simulink library "WECSim_Lib_Body_Elements"  (R2020b)
settings: Solver=VariableStepAuto  StartTime=0.0  StopTime=10.0  RelTol=1e-3
undefined symbols (not defined in the file or in its folder): body, simu, waves, X, Y, Z
libraries: nesl_utility x22, sm_lib x16, $bdroot x9, vrlib x3
(part 4 of 5)

== system WECSim_Lib_Body_Elements/Rigid Body/Hydrodynamic Body/Hydrostatic Restoring Force Calculation/Linear and Nonlinear Restoring Force Variant Subsystem/Linear Hydrostatic Restoring Force ==
  note: The total hydrostatic restoring force is due to a linear stiffness, the vertical buoyancy force (gravity - buoyancy) and a rotational buoyancy force if the center of gravity is not aligned with the center of buoyancy.
      |
      | F_restoring = F_linearRestoringStiffness + F_NetBuoyancy
      |
      | F_linear restoring = hydrostatic restoring coefficient * displacement
      | F_NetBuoyancy = F_gravity - F_buoyancy + F_rotational_buoyancy
      |
      | F_rotational_buoyancy = (cb-cg) x F_buoyancy
      | F_buoyancy = rho*g*V_0
      | F_gravity = m*g
  In1 : Inport
  Add : Sum
  Bus Selector : BusSelector  OutputSignals=mass,volume,centerBuoyancy,linearHydroRestCoef
  Net Buoyancy Force : Subsystem
  Product2 : Product  Multiplication=Matrix(*)
  Out1 : Outport
  wires:
  In1/1 -> Product2/2  "x"
  Bus Selector/4 -> Product2/1  "<linearHydroRestCoef>"
  Add/1 -> Out1/1  "F_Restoring"
  Product2/1 -> Add/2  "Linear Restoring Force"
  Net Buoyancy Force/1(F_NetBuoyancy) -> Add/1  "Net buoyancy force"
  [body1_hydroForce] -> Bus Selector/1
  Bus Selector/3 -> Net Buoyancy Force/3(Center of Buoyancy)  "<centerBuoyancy>"
  Bus Selector/2 -> Net Buoyancy Force/2(Volume)  "<volume>"
  Bus Selector/1 -> Net Buoyancy Force/1(Body Mass)  "<mass>"

== system WECSim_Lib_Body_Elements/Rigid Body/Hydrodynamic Body/Hydrostatic Restoring Force Calculation/Linear and Nonlinear Restoring Force Variant Subsystem/Nonlinear Hydrostatic Restoring Force ==
  In1 : Inport
  In2 : Inport  Port=2
  Bus Selector : BusSelector  OutputSignals=mass
  Center of Gravity : Constant  Value=body.centerGravity
  Gravity2 : Constant  Value=simu.gravity
  Rate Transition : RateTransition
  Rate Transition1 : RateTransition
  Restoring Forces : MATLAB Function  TreatAsAtomicUnit=on  SystemSampleTime=simu.nonlinearDt
  STL areas : Constant  Value=body.geometry.area
  STL centers : Constant  Value=body.geometry.center
  STL normal vectors : Constant  Value=body.geometry.norm
  To Workspace1 : ToWorkspace  VariableName=body1_hspressure_out  SaveFormat=Structure With Time  SampleTime=-1
      settings: Decimation=round(simu.dtOut/simu.dt,0)
  Water Density1 : Constant  Value=simu.rho
  Out1 : Outport
  wires:
  In1/1 -> Restoring Forces/1(x)
  Center of Gravity/1 -> Restoring Forces/8(cg)
  Gravity2/1 -> Restoring Forces/7(g)  "g"
  Water Density1/1 -> Restoring Forces/6(rho)
  STL normal vectors/1 -> Restoring Forces/4(tnorm)
  STL centers/1 -> Restoring Forces/3(center)
  In2/1 -> Restoring Forces/2(elv)
  STL areas/1 -> Restoring Forces/5(area)
  Bus Selector/1 -> Restoring Forces/9(mass)  "<mass>"
  Restoring Forces/2(p) -> Rate Transition1/1
  Rate Transition1/1 -> To Workspace1/1
  Restoring Forces/1(f) -> Rate Transition/1
  Rate Transition/1 -> Out1/1
  [body1_hydroForce] -> Bus Selector/1

== system WECSim_Lib_Body_Elements/Rigid Body/Hydrodynamic Body/Morison Element and Viscous Damping Force Calculation/Morison Element Variant Subsystem/Morison Element Off ==
  Constant : Constant  Value=zeros(1,body.dof)
  morison_force : Outport
  wires:
  Constant/1 -> morison_force/1

== system WECSim_Lib_Body_Elements/Rigid Body/Hydrodynamic Body/Morison Element and Viscous Damping Force Calculation/Morison Element Variant Subsystem/Morison Element On ==
  note: Chooses the appropriate Morison element variant dependent on the wave type. Note that if passive yaw is used, no block is chosen.
      |
      | If wave.type == 'noWave' | 'noWaveCIC' use No Wave Morison element
      | If wave.type == 'regularWave' | 'regularWaveCIC' use Regular Wave Morison element
      | If wave.type == 'irregularWave' or 'spectrumImport' use Irregular Wave Morison element
  note: 1) Add Subsystem or Model blocks as valid variant choices.
      | 2) You cannot connect blocks at this level. At simulation, connectivity is automatically
      | determined, based on the active variant and port name matching.
  displacement : Inport
  velocity : Inport  Port=2
  acceleration : Inport  Port=3
  time : Inport  Port=4
  Irregular Wave Morison Force : Subsystem  TreatAsAtomicUnit=on  SystemSampleTime=simu.morisonDt  VariantControl=sv_irregularWaves_b1
  No Wave Morison Force : Subsystem  VariantControl=sv_noWave
  Regular Wave Morison Force : Subsystem  TreatAsAtomicUnit=on  SystemSampleTime=simu.morisonDt  VariantControl=sv_regularWaves_b1
  morison_force : Outport

== system WECSim_Lib_Body_Elements/Rigid Body/Hydrodynamic Body/Nonlinear Wave Elevation/Linear or Instantaneous Free Surface/Instantaneous Water Free Surface ==
  note: Calculate the instantaneous wave elevation for the nonlinear hydrodynamics options.
  In1 : Inport
  In2 : Inport  Port=2
  Center of Gravity : Constant  Value=body.centerGravity
  Frequency Spacing : Constant  Value=waves.dOmega
  Instantaneous FS : MATLAB Function  TreatAsAtomicUnit=on
  Ramp Time : Constant  Value=simu.rampTime
  STL Centers : Constant  Value=body.geometry.center
  Wave Amplitude : Constant  Value=waves.amplitude
  Wave Direction : Constant  Value=waves.direction
  Wave Frequency : Constant  Value=waves.omega
  Wave Number : Constant  Value=waves.wavenumber
  Wave Random Phase : Constant  Value=waves.phase
  Wave Spread : Constant  Value=waves.spread
  Wave Type Number : Constant  Value=waves.typeNum
  Out1 : Outport
  wires:
  Instantaneous FS/1(f) -> Out1/1
  STL Centers/1 -> Instantaneous FS/2(center)
  Center of Gravity/1 -> Instantaneous FS/3(cg)
  Wave Number/1 -> Instantaneous FS/7(k)
  Wave Frequency/1 -> Instantaneous FS/5(w)
  Wave Type Number/1 -> Instantaneous FS/8(typeNum)
  Ramp Time/1 -> Instantaneous FS/10(rampT)
  Wave Random Phase/1 -> Instantaneous FS/11(phaseRand)
  Frequency Spacing/1 -> Instantaneous FS/6(dw)
  In2/1 -> Instantaneous FS/9(t)
  In1/1 -> Instantaneous FS/1(x)
  Wave Direction/1 -> Instantaneous FS/12(waveDir)
  Wave Amplitude/1 -> Instantaneous FS/4(AH)
  Wave Spread/1 -> Instantaneous FS/13(spread)

== system WECSim_Lib_Body_Elements/Rigid Body/Hydrodynamic Body/Nonlinear Wave Elevation/Linear or Instantaneous Free Surface/Mean Water Free Surface ==
  note: The mean water surface is always zero.
  zero : Constant  Value=0
  Out1 : Outport
  wires:
  zero/1 -> Out1/1

== system WECSim_Lib_Body_Elements/Rigid Body/Hydrodynamic Body/Variable Hydrodynamics Control/Variable Hydrodynamics Subsystem/noVariableHydro ==
  all_hydroForce : Inport
  Bus Selector : BusSelector  OutputSignals=hf1
  selected_hydroForce : Outport
  wires:
  Bus Selector/1 -> selected_hydroForce/1  "<hf1>"
  all_hydroForce/1 -> Bus Selector/1  "x"

== system WECSim_Lib_Body_Elements/Rigid Body/Hydrodynamic Body/Variable Hydrodynamics Control/Variable Hydrodynamics Subsystem/variableHydro ==
  all_hydroForce : Inport
  Bus Selector : BusSelector  OutputSignals=hf1
  Multiport Switch : MultiPortSwitch  Inputs=1  DataPortForDefault=Additional data port  DiagnosticForDefault=Warning  OutDataTypeStr=Inherit: Same as first data input  RndMeth=Round
      settings: LockScale=on
  To Workspace : ToWorkspace  VariableName=body1_hydroForceIndex  SaveFormat=Structure With Time  SampleTime=simu.dtOut
  selected_hydroForce : Outport
  wires:
  all_hydroForce/1 -> Bus Selector/1
  [body1_hydroForceIndex] -> To Workspace/1, Multiport Switch/1
  Multiport Switch/1 -> selected_hydroForce/1
  Bus Selector/1 -> Multiport Switch/2  "<hf1>"

== system WECSim_Lib_Body_Elements/Rigid Body/Hydrodynamic Body/Wave Diffraction and Excitation Force Calculation/Linear Wave Excitation Force Variant Subsystem/Irregular Wave Excitation Force ==
  note: Calculates the wave force, F_wave, for the case of Irregular Waves.
      |
      | The total force is the combination of the real excitation force, imaginary excitation force, and real part of the mean drift force (fExt.md)
      |
      | F_wave =   sum(A * cos(w * t) * Re{Fext(i)}
      |                            -  A * sin(w * t) * Im{Fext(i)}
      |                            + A * Re(Fext.md(i))
      |                            )
      |
      | where i = each frequency bin
  Time : Inport
  Displacement : Inport  Port=2
  body_hydroForce : Inport  Port=3
  Add : Sum  Inputs=+-
  Bus Selector : BusSelector  OutputSignals=fExt.re,fExt.im,fExt.md
  Center of Gravity : Constant  Value=body.centerGravity
  Constant : Constant  Value=zeros(1,body.dof-3)
  Displacement Phase Enable1 : Constant  Value=body.largeXYDisplacement.option
  Frequency Spacing Delta Omega : Constant  Value=Nwave.dOmega  VectorParams1D=off
  MATLAB Function : MATLAB Function  TreatAsAtomicUnit=on
  MATLAB Function2 : MATLAB Function  TreatAsAtomicUnit=on
  Mux : Mux  Inputs=2
  Random Phase : Constant  Value=Nwave.phase  VectorParams1D=off
  Selector : Selector  IndexOptions=Index vector (dialog)  Indices=[1 2]  OutputSizes=1
  Sum : Sum  Inputs=|++
  Wave Frequency : Constant  Value=Nwave.omega  VectorParams1D=off
  Wave Frequency1 : Constant  Value=Nwave.omega  VectorParams1D=off
  Wave Number1 : Constant  Value=Nwave.wavenumber
  Wave Spectrum : Constant  Value=Nwave.amplitude  VectorParams1D=off
  Wave direction spread : Constant  Value=Nwave.spread  VectorParams1D=off
  Wave direction1 : Constant  Value=Nwave.direction  VectorParams1D=off
  Linear Excitation : Outport
  wires:
  MATLAB Function/1(Fext) -> Linear Excitation/1
  Wave Frequency/1 -> MATLAB Function/2(w)
  Bus Selector/2 -> MATLAB Function/4(fExtIM)  "<im>"
  Wave Spectrum/1 -> MATLAB Function/1(A)
  Time/1 -> MATLAB Function/7(time)
  Frequency Spacing Delta Omega/1 -> MATLAB Function/6(dw)
  Wave direction spread/1 -> MATLAB Function/9(spread)
  Bus Selector/3 -> MATLAB Function/10(fExtMD)  "<md>"
  MATLAB Function2/1(dispPhase) -> Sum/2
  Sum/1 -> MATLAB Function/5(phaseRand)
  Random Phase/1 -> Sum/1
  Wave Frequency1/1 -> MATLAB Function2/3(frequency)
  Displacement Phase Enable1/1 -> MATLAB Function2/2(enable)
  Selector/1 -> MATLAB Function2/1(disp)
  Displacement/1 -> Add/1  "t"
  Wave Number1/1 -> MATLAB Function2/4(wavenumber)
  Wave direction1/1 -> MATLAB Function/8(WaveDir), MATLAB Function2/5(direction)
  Bus Selector/1 -> MATLAB Function/3(fExtRE)  "<re>"
  body_hydroForce/1 -> Bus Selector/1
  Constant/1 -> Mux/2
  Mux/1 -> Add/2
  Center of Gravity/1 -> Mux/1  "cg"
  Add/1 -> Selector/1  "x_cg"

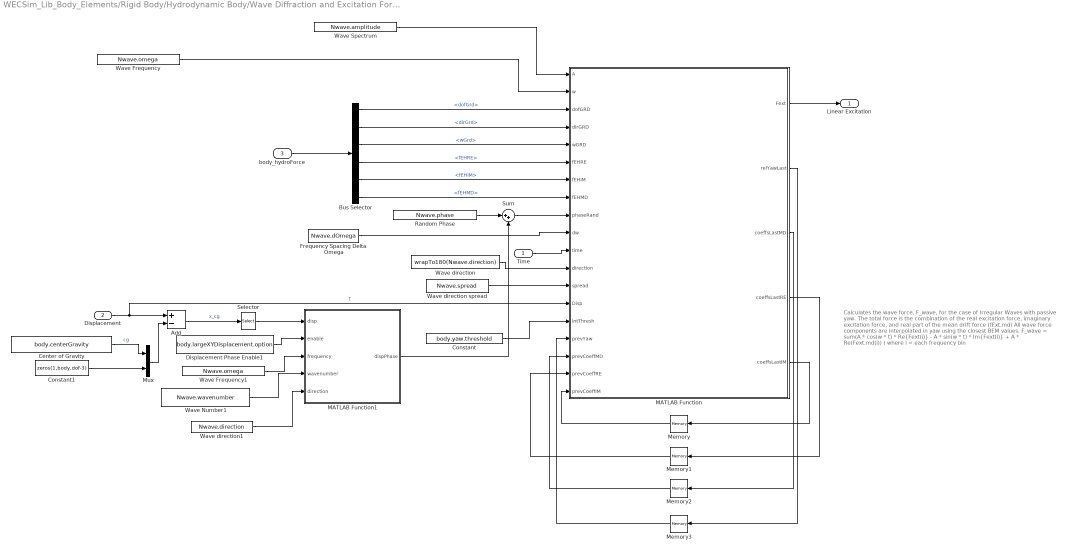
== system WECSim_Lib_Body_Elements/Rigid Body/Hydrodynamic Body/Wave Diffraction and Excitation Force Calculation/Linear Wave Excitation Force Variant Subsystem/Irregular Wave NonLinearYaw ==
  note: Calculates the wave force, F_wave, for the case of Irregular Waves with passive yaw.
      |
      | The total force is the combination of the real excitation force, imaginary excitation force, and real part of the mean drift force (fExt.md)
      |
      | All wave force components are interpolated in yaw using the closest BEM values.
      |
      | F_wave =   sum(A * cos(w * t) * Re{Fext(i)}
      |                            -  A * sin(w * t) * Im{Fext(i)}
      |                            + A * Re(Fext.md(i))
      |                            )
      |
      | where i = each frequency bin
  Time : Inport
  Displacement : Inport  Port=2
  body_hydroForce : Inport  Port=3
  Add : Sum  Inputs=+-
  Bus Selector : BusSelector  OutputSignals=fExt.dofGrd,fExt.dirGrd,fExt.wGrd,fExt.fEHRE,fExt.fEHIM,fExt.fEHMD
  Center of Gravity : Constant  Value=body.centerGravity
  Constant : Constant  Value=body.yaw.threshold
  Constant1 : Constant  Value=zeros(1,body.dof-3)
  Displacement Phase Enable1 : Constant  Value=body.largeXYDisplacement.option
  Frequency Spacing Delta Omega : Constant  Value=Nwave.dOmega  VectorParams1D=off
  MATLAB Function : MATLAB Function  TreatAsAtomicUnit=on
  MATLAB Function1 : MATLAB Function  TreatAsAtomicUnit=on
  Memory{,1..3} (4 alike) : Memory  InheritSampleTime=on  LinearizeAsDelay=on
  Mux : Mux  Inputs=2
  Random Phase : Constant  Value=Nwave.phase  VectorParams1D=off
  Selector : Selector  IndexOptions=Index vector (dialog)  Indices=[1 2]  OutputSizes=1
  Sum : Sum  Inputs=|++
  Wave Frequency : Constant  Value=Nwave.omega  VectorParams1D=off
  Wave Frequency1 : Constant  Value=Nwave.omega  VectorParams1D=off
  Wave Number1 : Constant  Value=Nwave.wavenumber
  Wave Spectrum : Constant  Value=Nwave.amplitude  VectorParams1D=off
  Wave direction : Constant  Value=wrapTo180(Nwave.direction)  VectorParams1D=off
  Wave direction spread : Constant  Value=Nwave.spread  VectorParams1D=off
  Wave direction1 : Constant  Value=Nwave.direction  VectorParams1D=off
  Linear Excitation : Outport
  wires:
  MATLAB Function/1(Fext) -> Linear Excitation/1
  Memory1/1 -> MATLAB Function/18(prevCoeffRE)
  MATLAB Function/4(coeffsLastRE) -> Memory1/1
  MATLAB Function/2(relYawLast) -> Memory3/1
  Memory2/1 -> MATLAB Function/17(prevCoeffMD)
  Bus Selector/3 -> MATLAB Function/5(wGRD)  "<wGrd>"
  Bus Selector/2 -> MATLAB Function/4(dirGRD)  "<dirGrd>"
  Frequency Spacing Delta Omega/1 -> MATLAB Function/10(dw)
  Wave direction/1 -> MATLAB Function/12(direction)
  MATLAB Function/5(coeffsLastIM) -> Memory/1
  Memory3/1 -> MATLAB Function/16(prevYaw)
  Constant/1 -> MATLAB Function/15(intThresh)
  MATLAB Function/3(coeffsLastMD) -> Memory2/1
  Bus Selector/4 -> MATLAB Function/6(fEHRE)  "<fEHRE>"
  Memory/1 -> MATLAB Function/19(prevCoeffIM)
  Wave Frequency/1 -> MATLAB Function/2(w)
  Wave Spectrum/1 -> MATLAB Function/1(A)
  Bus Selector/6 -> MATLAB Function/8(fEHMD)  "<fEHMD>"
  Wave direction spread/1 -> MATLAB Function/13(spread)
  Time/1 -> MATLAB Function/11(time)
  Random Phase/1 -> Sum/1
  Sum/1 -> MATLAB Function/9(phaseRand)
  Wave Frequency1/1 -> MATLAB Function1/3(frequency)
  Displacement Phase Enable1/1 -> MATLAB Function1/2(enable)
  Selector/1 -> MATLAB Function1/1(disp)
  Displacement/1 -> MATLAB Function/14(Disp), Add/1  "t"
  Wave Number1/1 -> MATLAB Function1/4(wavenumber)
  Wave direction1/1 -> MATLAB Function1/5(direction)
  MATLAB Function1/1(dispPhase) -> Sum/2
  body_hydroForce/1 -> Bus Selector/1
  Bus Selector/1 -> MATLAB Function/3(dofGRD)  "<dofGrd>"
  Bus Selector/5 -> MATLAB Function/7(fEHIM)  "<fEHIM>"
  Constant1/1 -> Mux/2
  Mux/1 -> Add/2
  Center of Gravity/1 -> Mux/1  "cg"
  Add/1 -> Selector/1  "x_cg"

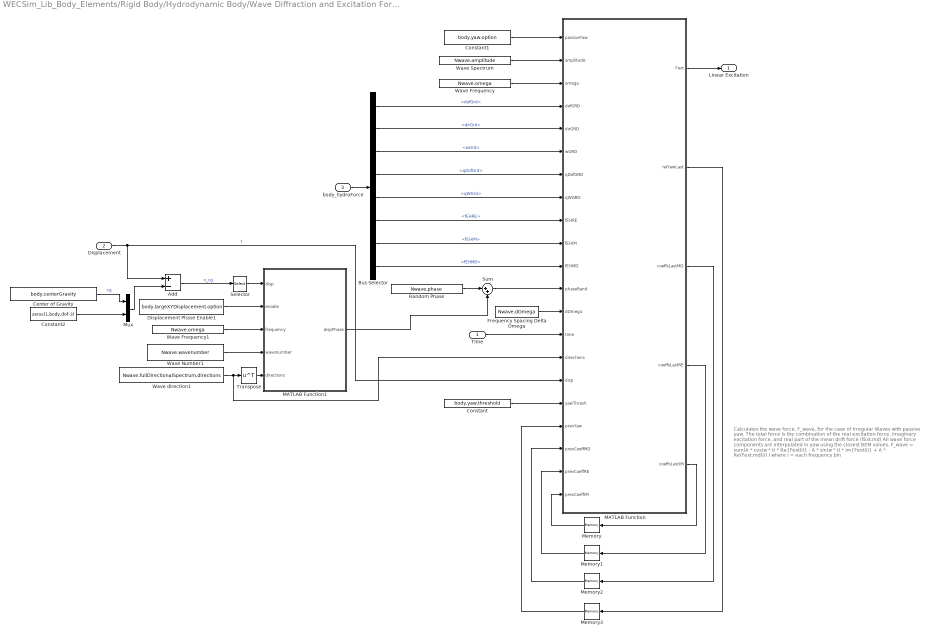
== system WECSim_Lib_Body_Elements/Rigid Body/Hydrodynamic Body/Wave Diffraction and Excitation Force Calculation/Linear Wave Excitation Force Variant Subsystem/Irregular Wave Full Direction ==
  note: Calculates the wave force, F_wave, for the case of Irregular Waves with passive yaw.
      |
      | The total force is the combination of the real excitation force, imaginary excitation force, and real part of the mean drift force (fExt.md)
      |
      | All wave force components are interpolated in yaw using the closest BEM values.
      |
      | F_wave =   sum(A * cos(w * t) * Re{Fext(i)}
      |                            -  A * sin(w * t) * Im{Fext(i)}
      |                            + A * Re(Fext.md(i))
      |                            )
      |
      | where i = each frequency bin
  Time : Inport
  Displacement : Inport  Port=2
  body_hydroForce : Inport  Port=3
  Add : Sum  Inputs=+-
  Bus Selector : BusSelector  OutputSignals=fExt.dofGrd,fExt.dirGrd,fExt.wGrd,fExt.qDofGrd,fExt.qWGrd,fExt.fEHRE,fExt.fEHIM,fExt.fEHMD
  Center of Gravity : Constant  Value=body.centerGravity
  Constant : Constant  Value=body.yaw.threshold
  Constant1 : Constant  Value=body.yaw.option
  Constant2 : Constant  Value=zeros(1,body.dof-3)
  Displacement Phase Enable1 : Constant  Value=body.largeXYDisplacement.option
  Frequency Spacing Delta Omega : Constant  Value=Nwave.dOmega  VectorParams1D=off
  MATLAB Function : MATLAB Function  TreatAsAtomicUnit=on
  MATLAB Function1 : MATLAB Function  TreatAsAtomicUnit=on
  Memory : Memory  InitialCondition=zeros(length(Nwave.fullDirectionalSpectrum.directions),length(Nwave.omega),6)  InheritSampleTime=on  LinearizeAsDelay=on
  Memory1 : Memory  InitialCondition=zeros(length(Nwave.fullDirectionalSpectrum.directions),length(Nwave.omega),6)  InheritSampleTime=on  LinearizeAsDelay=on
  Memory2 : Memory  InitialCondition=zeros(length(Nwave.fullDirectionalSpectrum.directions),length(Nwave.omega),6)  InheritSampleTime=on  LinearizeAsDelay=on
  Memory3 : Memory  InitialCondition=zeros(size(Nwave.fullDirectionalSpectrum.directions))  InheritSampleTime=on  LinearizeAsDelay=on
  Mux : Mux  Inputs=2
  Random Phase : Constant  Value=Nwave.phase  VectorParams1D=off
  Selector : Selector  IndexOptions=Index vector (dialog)  Indices=[1 2]  OutputSizes=1
  Sum : Sum  Inputs=|++
  Transpose : Math  Operator=transpose  SaturateOnIntegerOverflow=on
  Wave Frequency : Constant  Value=Nwave.omega  VectorParams1D=off
  Wave Frequency1 : Constant  Value=Nwave.omega  VectorParams1D=off
  Wave Number1 : Constant  Value=Nwave.wavenumber
  Wave Spectrum : Constant  Value=Nwave.amplitude  VectorParams1D=off
  Wave direction1 : Constant  Value=Nwave.fullDirectionalSpectrum.directions  VectorParams1D=off
  Linear Excitation : Outport
  wires:
  Constant1/1 -> MATLAB Function/1(passiveYaw)
  MATLAB Function/3(coeffsLastMD) -> Memory2/1
  MATLAB Function/4(coeffsLastRE) -> Memory1/1
  Wave direction1/1 -> MATLAB Function/15(directions), Transpose/1
  Displacement Phase Enable1/1 -> MATLAB Function1/2(enable)
  Selector/1 -> MATLAB Function1/1(disp)
  Wave Frequency1/1 -> MATLAB Function1/3(frequency)
  MATLAB Function/1(Fext) -> Linear Excitation/1
  Sum/1 -> MATLAB Function/12(phaseRand)
  Wave Spectrum/1 -> MATLAB Function/2(amplitude)
  Memory1/1 -> MATLAB Function/20(prevCoeffRE)
  Memory/1 -> MATLAB Function/21(prevCoeffIM)
  Frequency Spacing Delta Omega/1 -> MATLAB Function/13(dOmega)
  MATLAB Function/5(coeffsLastIM) -> Memory/1
  Time/1 -> MATLAB Function/14(time)
  Constant/1 -> MATLAB Function/17(yawThresh)
  Memory3/1 -> MATLAB Function/18(prevYaw)
  Memory2/1 -> MATLAB Function/19(prevCoeffMD)
  Wave Number1/1 -> MATLAB Function1/4(wavenumber)
  MATLAB Function/2(relYawLast) -> Memory3/1
  Bus Selector/7 -> MATLAB Function/10(fEHIM)  "<fEHIM>"
  Bus Selector/3 -> MATLAB Function/6(wGRD)  "<wGrd>"
  body_hydroForce/1 -> Bus Selector/1
  Bus Selector/1 -> MATLAB Function/4(dofGRD)  "<dofGrd>"
  Bus Selector/6 -> MATLAB Function/9(fEHRE)  "<fEHRE>"
  Bus Selector/8 -> MATLAB Function/11(fEHMD)  "<fEHMD>"
  Bus Selector/2 -> MATLAB Function/5(dirGRD)  "<dirGrd>"
  Bus Selector/4 -> MATLAB Function/7(qDofGRD)  "<qDofGrd>"
  Bus Selector/5 -> MATLAB Function/8(qWGRD)  "<qWGrd>"
  MATLAB Function1/1(dispPhase) -> Sum/2
  Random Phase/1 -> Sum/1
  Constant2/1 -> Mux/2
  Mux/1 -> Add/2
  Center of Gravity/1 -> Mux/1  "cg"
  Displacement/1 -> MATLAB Function/16(disp), Add/1  "t"
  Add/1 -> Selector/1  "x_cg"
  Wave Frequency/1 -> MATLAB Function/3(omega)
  Transpose/1 -> MATLAB Function1/5(directions)

== system WECSim_Lib_Body_Elements/Rigid Body/Hydrodynamic Body/Wave Diffraction and Excitation Force Calculation/Linear Wave Excitation Force Variant Subsystem/No Wave Excitation Force ==
  Constant : Constant  Value=zeros(1,body.dof)
  Linear Excitation : Outport
  wires:
  Constant/1 -> Linear Excitation/1

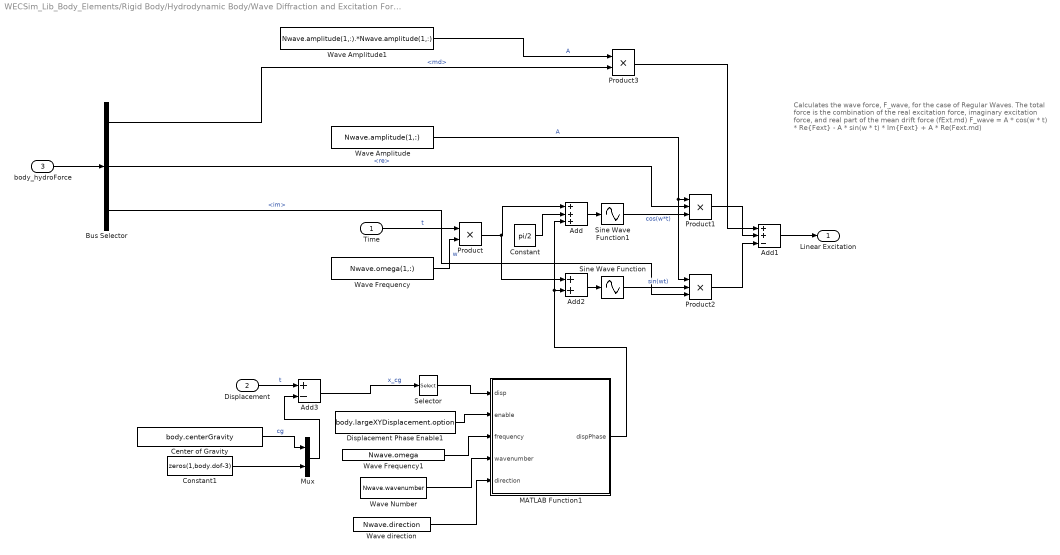
== system WECSim_Lib_Body_Elements/Rigid Body/Hydrodynamic Body/Wave Diffraction and Excitation Force Calculation/Linear Wave Excitation Force Variant Subsystem/Regular Wave Excitation Force ==
  note: Calculates the wave force, F_wave, for the case of Regular Waves.
      |
      | The total force is the combination of the real excitation force, imaginary excitation force, and real part of the mean drift force (fExt.md)
      |
      | F_wave =   A * cos(w * t) * Re{Fext}
      |                -  A * sin(w * t) * Im{Fext}
      |                + A * Re(Fext.md)
  Time : Inport
  Displacement : Inport  Port=2
  body_hydroForce : Inport  Port=3
  Add : Sum  Inputs=+++
  Add1 : Sum  Inputs=++-
  Add2 : Sum
  Add3 : Sum  Inputs=+-
  Bus Selector : BusSelector  OutputSignals=fExt.md,fExt.re,fExt.im
  Center of Gravity : Constant  Value=body.centerGravity
  Constant : Constant  Value=pi/2
  Constant1 : Constant  Value=zeros(1,body.dof-3)
  Displacement Phase Enable1 : Constant  Value=body.largeXYDisplacement.option
  MATLAB Function1 : MATLAB Function  TreatAsAtomicUnit=on
  Mux : Mux  Inputs=2
  Product : Product
  Product1 : Product  Inputs=3
  Product2 : Product  Inputs=3
  Product3 : Product
  Selector : Selector  IndexOptions=Index vector (dialog)  Indices=[1 2]  OutputSizes=1
  Sine Wave Function : Sin  TimeSource=Use external signal  SampleTime=0
  Sine Wave Function1 : Sin  TimeSource=Use external signal  SampleTime=0
  Wave Amplitude : Constant  Value=Nwave.amplitude(1,:)
  Wave Amplitude1 : Constant  Value=Nwave.amplitude(1,:).*Nwave.amplitude(1,:)
  Wave Frequency : Constant  Value=Nwave.omega(1,:)
  Wave Frequency1 : Constant  Value=Nwave.omega  VectorParams1D=off
  Wave Number : Constant  Value=Nwave.wavenumber
  Wave direction : Constant  Value=Nwave.direction  VectorParams1D=off
  Linear Excitation : Outport
  wires:
  Time/1 -> Product/1  "t"
  Wave Frequency/1 -> Product/2  "w"
  Product/1 -> Add2/1, Add/1
  Sine Wave Function1/1 -> Product1/3  "cos(w*t)"
  Sine Wave Function/1 -> Product2/2  "sin(wt)"
  Product1/1 -> Add1/2
  Product2/1 -> Add1/3
  Add1/1 -> Linear Excitation/1
  Wave Amplitude/1 -> Product2/1, Product1/1  "A"
  Add/1 -> Sine Wave Function1/1
  Constant/1 -> Add/2
  Wave Amplitude1/1 -> Product3/1  "A"
  Product3/1 -> Add1/1
  Displacement/1 -> Add3/1  "t"
  Displacement Phase Enable1/1 -> MATLAB Function1/2(enable)
  MATLAB Function1/1(dispPhase) -> Add/3, Add2/2
  Add2/1 -> Sine Wave Function/1
  Selector/1 -> MATLAB Function1/1(disp)
  Wave Frequency1/1 -> MATLAB Function1/3(frequency)
  Wave Number/1 -> MATLAB Function1/4(wavenumber)
  Wave direction/1 -> MATLAB Function1/5(direction)
  body_hydroForce/1 -> Bus Selector/1
  Bus Selector/1 -> Product3/2  "<md>"
  Bus Selector/2 -> Product1/2  "<re>"
  Bus Selector/3 -> Product2/3  "<im>"
  Constant1/1 -> Mux/2
  Mux/1 -> Add3/2
  Center of Gravity/1 -> Mux/1  "cg"
  Add3/1 -> Selector/1  "x_cg"

== system WECSim_Lib_Body_Elements/Rigid Body/Hydrodynamic Body/Wave Diffraction and Excitation Force Calculation/Linear Wave Excitation Force Variant Subsystem/Regular Wave NonLinear Yaw ==
  note: Calculates the wave force, F_wave, for the case of Regular Waves with passive yaw.
      |
      | The total force is the combination of the real excitation force, imaginary excitation force, and real part of the mean drift force (fExt.md)
      |
      | All wave force components are interpolated in yaw using the closest BEM values.
      |
      | F_wave =   A * cos(w * t) * Re{Fext}
      |                -  A * sin(w * t) * Im{Fext}
      |                + A * Re(Fext.md)
  Time : Inport
  Displacement : Inport  Port=2
  body_hydroForce : Inport  Port=3
  Add : Sum  Inputs=+-
  Bus Selector : BusSelector  OutputSignals=fExt.dofGrd,fExt.dirGrd,fExt.fEHRE,fExt.fEHIM,fExt.fEHMD
  Center of Gravity : Constant  Value=body.centerGravity
  Constant : Constant  Value=body.yaw.threshold
  Constant1 : Constant  Value=zeros(1,body.dof-3)
  Displacement Phase Enable1 : Constant  Value=body.largeXYDisplacement.option
  MATLAB Function1 : MATLAB Function  TreatAsAtomicUnit=on
  MATLAB Function3 : MATLAB Function  TreatAsAtomicUnit=on
  Memory{,1..3} (4 alike) : Memory  InheritSampleTime=on  LinearizeAsDelay=on
  Mux : Mux  Inputs=2
  Selector : Selector  IndexOptions=Index vector (dialog)  Indices=[1 2]  OutputSizes=1
  Wave Amplitude : Constant  Value=Nwave.amplitude(1,:)
  Wave Frequency : Constant  Value=Nwave.omega(1,:)
  Wave Frequency1 : Constant  Value=Nwave.omega  VectorParams1D=off
  Wave Number1 : Constant  Value=Nwave.wavenumber
  Wave direction : Constant  Value=wrapTo180(Nwave.direction)  VectorParams1D=off
  Wave direction1 : Constant  Value=Nwave.direction  VectorParams1D=off
  Linear Excitation : Outport
  wires:
  Memory2/1 -> MATLAB Function1/14(prevCoeffMD)
  Constant/1 -> MATLAB Function1/11(intThresh)
  Bus Selector/2 -> MATLAB Function1/4(dirGRD)  "<dirGrd>"
  Memory1/1 -> MATLAB Function1/15(prevCoeffRE)
  Wave direction/1 -> MATLAB Function1/9(WaveDir)
  MATLAB Function1/3(coeffsLastMD) -> Memory2/1
  Wave Amplitude/1 -> MATLAB Function1/1(A)  "A"
  Memory/1 -> MATLAB Function1/16(prevCoeffIM)
  Bus Selector/5 -> MATLAB Function1/7(fEHMD)  "<fEHMD>"
  Memory3/1 -> MATLAB Function1/13(prevYaw)
  MATLAB Function1/4(coeffsLastRE) -> Memory1/1
  MATLAB Function1/2(relYawLast) -> Memory3/1
  MATLAB Function1/5(coeffsLastIM) -> Memory/1
  Wave Frequency/1 -> MATLAB Function1/2(w)  "w"
  MATLAB Function1/1(Fext) -> Linear Excitation/1
  Time/1 -> MATLAB Function1/8(time)
  MATLAB Function3/1(dispPhase) -> MATLAB Function1/12(phase)
  Wave direction1/1 -> MATLAB Function3/5(direction)
  Displacement/1 -> MATLAB Function1/10(Disp), Add/1  "t"
  Wave Number1/1 -> MATLAB Function3/4(wavenumber)
  Displacement Phase Enable1/1 -> MATLAB Function3/2(enable)
  Selector/1 -> MATLAB Function3/1(disp)
  Wave Frequency1/1 -> MATLAB Function3/3(frequency)
  body_hydroForce/1 -> Bus Selector/1
  Bus Selector/1 -> MATLAB Function1/3(dofGRD)  "<dofGrd>"
  Bus Selector/4 -> MATLAB Function1/6(fEHIM)  "<fEHIM>"
  Bus Selector/3 -> MATLAB Function1/5(fEHRE)  "<fEHRE>"
  Constant1/1 -> Mux/2
  Mux/1 -> Add/2
  Center of Gravity/1 -> Mux/1  "cg"
  Add/1 -> Selector/1  "x_cg"

== system WECSim_Lib_Body_Elements/Rigid Body/Hydrodynamic Body/Wave Diffraction and Excitation Force Calculation/Linear Wave Excitation Force Variant Subsystem/User Defined Wave Excitation Force ==
  note: Calculates the wave force, F_wave, for the case of User Defined Waves.
      |
      | F_wave = convolution calculation [1x6]
  InputWaveForceTimeHistory1 : FromWorkspace  VariableName=[Nwave.waveAmpTime(:,1),body.hydroForce.hf1.userDefinedFe]
  Linear Excitation : Outport
  wires:
  InputWaveForceTimeHistory1/1 -> Linear Excitation/1

== system WECSim_Lib_Body_Elements/Rigid Body/Hydrodynamic Body/Wave Diffraction and Excitation Force Calculation/Nonlinear FK Force Variant Subsystem/No Nonlinear FroudeKrylov Force ==
  Constant : Constant  Value=zeros(1,body.dof)
  Nonlinear Excitation : Outport
  wires:
  Constant/1 -> Nonlinear Excitation/1

== system WECSim_Lib_Body_Elements/Rigid Body/Hydrodynamic Body/Wave Diffraction and Excitation Force Calculation/Nonlinear FK Force Variant Subsystem/With Nonlinear FroudeKrylov Force ==
  Time : Inport
  Displacement : Inport  Port=2
  WaveElv : Inport  Port=3
  Add : Sum  Inputs=+-
  Center of Gravity : Constant  Value=body.hydroData(1).properties.centerGravity
  Center of Gravity1 : Constant  Value=body.hydroData(1).properties.centerGravity
  Constant : Constant  Value=zeros(1,body.dof-3)
  Deep Water Flag : Constant  Value=waves.deepWater
  Diffraction and Excitation Forces : MATLAB Function  TreatAsAtomicUnit=on
  Frequency Spacing : Constant  Value=waves.dOmega
  Gravity : Constant  Value=simu.gravity
  Mux : Mux  Inputs=2
  STL Areas : Constant  Value=body.geometry.area
  STL Centers : Constant  Value=body.geometry.center
  STL Normal Vectors : Constant  Value=body.geometry.norm
  To Workspace : ToWorkspace  VariableName=body1_wavenonlinearpressure_out  SaveFormat=Structure With Time  SampleTime=-1
      settings: Decimation=round(simu.dtOut/simu.dt,0)
  To Workspace1 : ToWorkspace  VariableName=body1_wavelinearpressure_out  SaveFormat=Structure With Time  SampleTime=-1
      settings: Decimation=round(simu.dtOut/simu.dt,0)
  Water Density : Constant  Value=simu.rho
  Water Depth : Constant  Value=waves.waterDepth
  Wave Amplitude : Constant  Value=waves.amplitude
  Wave Direction : Constant  Value=waves.direction
  Wave Frequency : Constant  Value=waves.omega
  Wave Number : Constant  Value=waves.wavenumber
  Wave Random Phase : Constant  Value=waves.phase
  Wave Spread : Constant  Value=waves.spread
  Wave Type Number : Constant  Value=waves.typeNum
  Nonlinear Excitation : Outport
  wires:
  Center of Gravity1/1 -> Diffraction and Excitation Forces/10(cg)
  Diffraction and Excitation Forces/1(f) -> Nonlinear Excitation/1
  Gravity/1 -> Diffraction and Excitation Forces/9(g)
  Water Density/1 -> Diffraction and Excitation Forces/8(rho)
  STL Normal Vectors/1 -> Diffraction and Excitation Forces/6(tnorm)
  WaveElv/1 -> Diffraction and Excitation Forces/2(elv)
  Time/1 -> Diffraction and Excitation Forces/18(t)
  Wave Amplitude/1 -> Diffraction and Excitation Forces/11(AH)
  Wave Frequency/1 -> Diffraction and Excitation Forces/12(w)
  Frequency Spacing/1 -> Diffraction and Excitation Forces/13(dw)
  Wave Type Number/1 -> Diffraction and Excitation Forces/17(typeNum)
  Wave Number/1 -> Diffraction and Excitation Forces/16(k)
  Water Depth/1 -> Diffraction and Excitation Forces/14(wDepth)
  Wave Random Phase/1 -> Diffraction and Excitation Forces/19(phaseRand)
  Deep Water Flag/1 -> Diffraction and Excitation Forces/15(deepWater)
  Add/1 -> Diffraction and Excitation Forces/1(x)  "x_cg"
  Mux/1 -> Add/2
  Center of Gravity/1 -> Mux/1  "cg"
  Constant/1 -> Mux/2
  Displacement/1 -> Add/1
  Diffraction and Excitation Forces/3(wpMeanFS) -> To Workspace1/1
  Diffraction and Excitation Forces/2(wp) -> To Workspace/1
  STL Areas/1 -> Diffraction and Excitation Forces/7(area)
  Wave Direction/1 -> Diffraction and Excitation Forces/3(direction)
  STL Centers/1 -> Diffraction and Excitation Forces/5(center)
  Wave Spread/1 -> Diffraction and Excitation Forces/4(spread)

== system WECSim_Lib_Body_Elements/Rigid Body/Hydrodynamic Body/Wave Diffraction and Excitation Force Calculation/Second Order Excitation Force Variant Subsystem/No Second Order Excitation Force ==
  Constant : Constant  Value=zeros(1,body.dof)
  Second Order Excitation : Outport
  wires:
  Constant/1 -> Second Order Excitation/1

== system WECSim_Lib_Body_Elements/Rigid Body/Hydrodynamic Body/Wave Diffraction and Excitation Force Calculation/Second Order Excitation Force Variant Subsystem/With Second Order Excitation Force ==
  Time : Inport
  body_hydroForce : Inport  Port=2
  displacement : Inport  Port=3
  Bus Selector : BusSelector  OutputSignals=QTF.time,QTF.fFastVaryingForces,QTF.fSlowVaryingForces
  Diffraction and Excitation Forces : MATLAB Function
  Second Order Excitation : Outport
  wires:
  Diffraction and Excitation Forces/1(f) -> Second Order Excitation/1
  Time/1 -> Diffraction and Excitation Forces/4(t)
  body_hydroForce/1 -> Bus Selector/1
  Bus Selector/1 -> Diffraction and Excitation Forces/1(time_vector)  "<time>"
  Bus Selector/3 -> Diffraction and Excitation Forces/3(slowVaryingForce)  "<fSlowVaryingForces>"
  Bus Selector/2 -> Diffraction and Excitation Forces/2(fastVaryingForce)  "<fFastVaryingForces>"
  displacement/1 -> Diffraction and Excitation Forces/5(displacement)

== system WECSim_Lib_Body_Elements/Rigid Body/Hydrodynamic Body/Wave Radiation Forces Calculation/SS CI and Constant-Damping-CoeVariant Subsystem/Constant Coefficients ==
  note: F = damping * velocity
  velocity : Inport
  Bus Selector : BusSelector  OutputSignals=fDamping
  Product : Product  Multiplication=Matrix(*)
  Out1 : Outport
  wires:
  Product/1 -> Out1/1  "F_Single Frequency"
  velocity/1 -> Product/2
  [body1_hydroForce] -> Bus Selector/1
  Bus Selector/1 -> Product/1  "<fDamping>"

== system WECSim_Lib_Body_Elements/Rigid Body/Hydrodynamic Body/Wave Radiation Forces Calculation/SS CI and Constant-Damping-CoeVariant Subsystem/Convolution Integral Calculation ==
  velocity : Inport
  Convolution Variant Subsystem : Subsystem  Variant=on  VariantControl=Subsystem
  Reshape : Reshape
  Out1 : Outport
  wires:
  Reshape/1 -> Out1/1
  velocity/1 -> Convolution Variant Subsystem/1(velocity)
  Convolution Variant Subsystem/1(Frad) -> Reshape/1

== system WECSim_Lib_Body_Elements/Rigid Body/Hydrodynamic Body/Wave Radiation Forces Calculation/SS CI and Constant-Damping-CoeVariant Subsystem/FIR Filter Calculation ==
  velocity : Inport
  FIR Filter Matrix : Subsystem  mask{B2B=simu.b2b, body=body}
      mask prompts: body "bodyClass"
      mask init: same as WECSim_Lib_Body_Elements/Flex Body/Wave Radiation Forces Calculation/Wave Radiation Forces Calculation/SS CI and Constant-Damping-CoeVariant Subsystem/FIR Filter Calculation/FIR Filter Matrix
  Rate Transition : RateTransition  OutPortSampleTime=simu.cicDt
  Rate Transition1 : RateTransition  OutPortSampleTime=simu.cicDt
  Out1 : Outport
  wires:
  velocity/1 -> Rate Transition/1
  FIR Filter Matrix/1(Out1) -> Rate Transition1/1
  Rate Transition/1 -> FIR Filter Matrix/1(velocity)
  Rate Transition1/1 -> Out1/1

== system WECSim_Lib_Body_Elements/Rigid Body/Hydrodynamic Body/Wave Radiation Forces Calculation/SS CI and Constant-Damping-CoeVariant Subsystem/State-Space Calculation  ==
  note: Calculate the radiation damping based on the state space formulation. Coefficients are defined in body.hydroForce.ssRadf
  velocity : Inport
  State-Space : StateSpace  A=body.hydroForce.hf1.ssRadf.A  B=body.hydroForce.hf1.ssRadf.B  C=body.hydroForce.hf1.ssRadf.C  D=body.hydroForce.hf1.ssRadf.D  InitialCondition=0
  Out1 : Outport
  wires:
  velocity/1 -> State-Space/1  "x"
  State-Space/1 -> Out1/1

== system WECSim_Lib_Body_Elements/Flex Body/Hydrostatic Restoring Force Calculation/Hydrostatic Restoring Force Calculation/Linear and Nonlinear Restoring Force Variant Subsystem/Linear Hydrostatic Restoring Force/Net Buoyancy Force ==
  note: The total buoyancy force is due to the vertical buoyancy force (gravity - buoyancy) and a rotational buoyancy force if the center of gravity is not aligned with the center of buoyancy.
      |
      | F_NetBuoyancy = F_gravity - F_buoyancy + F_rotational_buoyancy
      |
      | F_rotational_buoyancy = (cb-cg) x F_buoyancy
      | F_buoyancy = rho*g*V_0
      | F_gravity = m*g
  Body Mass : Inport
  Volume : Inport  Port=2
  Center of Buoyancy : Inport  Port=3
  Add1 : Sum  Inputs=+-
  Add2 : Sum
  Add3 : Sum  Inputs=+-
  Assignment (Add Net Bouyancy Force to Z-Direction) : Assignment  IndexOptions=Index vector (dialog)  Indices=3  OutputSizes=1
  Assignment (Add Net Bouyancy Force to Z-Direction)1 : Assignment  IndexOptions=Index vector (dialog)  Indices=3  OutputSizes=1
  Assignment (Add Net Bouyancy Force to Z-Direction)2 : Assignment  IndexOptions=Index vector (dialog)  Indices=4:6  OutputSizes=1
  Center of Gravity : Constant  Value=body.centerGravity
  Constant1 : Constant  Value=zeros(1,body.dof)
  Constant2 : Constant  Value=[0 0 0]
  Cross Product : vrlib/Utilities/Cross Product
  Gravity : Constant  Value=simu.gravity
  Product : Product
  Product1 : Product  Inputs=3
  Water Density : Constant  Value=simu.rho
  F_NetBuoyancy : Outport
  wires:
  Center of Buoyancy/1 -> Add3/1  "cb"
  Volume/1 -> Product1/3  "V0"
  Add1/1 -> Assignment (Add Net Bouyancy Force to Z-Direction)/2
  Body Mass/1 -> Product/2  "m"
  Cross Product/1 -> Assignment (Add Net Bouyancy Force to Z-Direction)2/2
  Add2/1 -> F_NetBuoyancy/1  "Net buoyancy force"
  Add3/1 -> Cross Product/2
  Constant2/1 -> Assignment (Add Net Bouyancy Force to Z-Direction)1/1
  Center of Gravity/1 -> Add3/2  "cg"
  Constant1/1 -> Assignment (Add Net Bouyancy Force to Z-Direction)/1, Assignment (Add Net Bouyancy Force to Z-Direction)2/1
  Assignment (Add Net Bouyancy Force to Z-Direction)1/1 -> Cross Product/1
  Assignment (Add Net Bouyancy Force to Z-Direction)/1 -> Add2/1  "Vertical Buoyancy Force"
  Water Density/1 -> Product1/1  "rho"
  Gravity/1 -> Product/1, Product1/2  "g"
  Product1/1 -> Assignment (Add Net Bouyancy Force to Z-Direction)1/2, Add1/2  "F_Buoyancy"
  Product/1 -> Add1/1  "F_Gravity"
  Assignment (Add Net Bouyancy Force to Z-Direction)2/1 -> Add2/2  "Rotational buoyancy force"

== system WECSim_Lib_Body_Elements/Flex Body/Hydrostatic Restoring Force Calculation/Hydrostatic Restoring Force Calculation/Linear and Nonlinear Restoring Force Variant Subsystem/Nonlinear Hydrostatic Restoring Force/Net Buoyancy Force ==
  note: The total buoyancy force is due to the vertical buoyancy force (gravity - buoyancy) and a rotational buoyancy force if the center of gravity is not aligned with the center of buoyancy.
      |
      | F_NetBuoyancy = F_gravity - F_buoyancy + F_rotational_buoyancy
      |
      | F_rotational_buoyancy = (cb-cg) x F_buoyancy
      | F_buoyancy = rho*g*V_0
      | F_gravity = m*g
  Body Mass : Inport
  Volume : Inport  Port=2
  Center of Buoyancy : Inport  Port=3
  Add1 : Sum  Inputs=+-
  Add2 : Sum
  Add3 : Sum  Inputs=+-
  Assignment (Add Net Bouyancy Force to Z-Direction) : Assignment  IndexOptions=Index vector (dialog)  Indices=3  OutputSizes=1
  Assignment (Add Net Bouyancy Force to Z-Direction)1 : Assignment  IndexOptions=Index vector (dialog)  Indices=3  OutputSizes=1
  Assignment (Add Net Bouyancy Force to Z-Direction)2 : Assignment  IndexOptions=Index vector (dialog)  Indices=4:6  OutputSizes=1
  Center of Gravity : Constant  Value=body.centerGravity
  Constant1 : Constant  Value=zeros(1,body.dof)
  Constant2 : Constant  Value=[0 0 0]
  Cross Product : vrlib/Utilities/Cross Product
  Gravity : Constant  Value=simu.gravity
  Product : Product
  Product1 : Product  Inputs=3
  Water Density : Constant  Value=simu.rho
  F_NetBuoyancy : Outport
  wires:
  Center of Buoyancy/1 -> Add3/1  "cb"
  Volume/1 -> Product1/3  "V0"
  Add1/1 -> Assignment (Add Net Bouyancy Force to Z-Direction)/2
  Body Mass/1 -> Product/2  "m"
  Cross Product/1 -> Assignment (Add Net Bouyancy Force to Z-Direction)2/2
  Add2/1 -> F_NetBuoyancy/1  "Net buoyancy force"
  Add3/1 -> Cross Product/2
  Constant2/1 -> Assignment (Add Net Bouyancy Force to Z-Direction)1/1
  Center of Gravity/1 -> Add3/2  "cg"
  Constant1/1 -> Assignment (Add Net Bouyancy Force to Z-Direction)/1, Assignment (Add Net Bouyancy Force to Z-Direction)2/1
  Assignment (Add Net Bouyancy Force to Z-Direction)1/1 -> Cross Product/1
  Assignment (Add Net Bouyancy Force to Z-Direction)/1 -> Add2/1  "Vertical Buoyancy Force"
  Water Density/1 -> Product1/1  "rho"
  Gravity/1 -> Product/1, Product1/2  "g"
  Product1/1 -> Assignment (Add Net Bouyancy Force to Z-Direction)1/2, Add1/2  "F_Buoyancy"
  Product/1 -> Add1/1  "F_Gravity"
  Assignment (Add Net Bouyancy Force to Z-Direction)2/1 -> Add2/2  "Rotational buoyancy force"

== system WECSim_Lib_Body_Elements/Flex Body/Wave Radiation Forces Calculation/Wave Radiation Forces Calculation/SS CI and Constant-Damping-CoeVariant Subsystem/Convolution Integral Calculation/Convolution Variant Subsystem ==
  velocity : Inport
  Convolution Integral Calculation : Subsystem  VariantControl=sv_b1_noVariableHydro
  Convolution Integral Surface Calculation : Subsystem  VariantControl=sv_b1_variableHydro
  Frad : Outport

== system WECSim_Lib_Body_Elements/Flex Body/Wave Radiation Forces Calculation/Wave Radiation Forces Calculation/SS CI and Constant-Damping-CoeVariant Subsystem/FIR Filter Calculation/FIR Filter Matrix ==
  velocity : Inport
  FIR_filter_row : Subsystem  mask{body=body, B2B=simu.b2b, rowNo=1}
      mask prompts: body "BodyClass"
      mask init:
      | cb = gcb;
      | % The implementation that follows, calculates the radiation force, Fr, by
      | % calculating the Fr for each body mode by multiplying the velocity vector
      | % to the IRF matrix -- whose each row corresponds to the Fr for each of the
      | % modes corresponding to the velocity vector.
      | 
      | 
      | % Get the radiation IRF coefficients using body.hydroForce.irkb
      | set_param([cb '/Discrete FIR Filter'],...
      |            'position',[100, 0, 140, 180]);
      |          if rem(rowNo,6) ~= 0
      |         set_param([cb,'/Discrete FIR Filter'],...
      |                   'Coefficients', [sprintf('transpose(squeeze(body.hydroForce.hf1.irkb(:,%d,%d)))',rem(rowNo,6),1)]); 
      |          elseif rem(rowNo,6) == 0
      |         set_param([cb,'/Discrete FIR Filter'],...
      |                   'Coefficients', [sprintf('transpose(squeeze(body.hydroForce.hf1.irkb(:,%d,%d)))',6,1)]); 
      |          end
      | % Assign number of filters. The number of filter corresponds to the IRF
      | % matrix elements being used for the calculation for each row.
      | nFilt = body.dof + B2B*(body.total-1)*6;
      | 
      | % Add Demux channels corresponding to number of filters, and connect them to the corresponding filter.
      | 
      | set_param([cb '/Demux'],...
      |            'Outputs',sprintf('%d',nFilt));
      | try
      | add_line(cb,...
      |         'Demux/1',...
      |         ['Discrete FIR Filter','/1'], ...     
      |         'autorouting','on');
      | catch
      | end
      | 
      | try
      | add_line(cb,...
      |         'Discrete FIR Filter/1', ...     
      |         'Add/1',...
      |         'autorouting','on');
      | catch 
      | end
      | 
      | % Add filters 
      | 
      | for i = 2:nFilt
      | 
      |      try
      |         add_block([cb,'/Discrete FIR Filter'],[cb,'/Discrete FIR Filter ',num2str(i)],'MakeNameUnique','off',...
      |                    'Position',[100*i, 0, 40+100*i, 180],'BackgroundColor','white');
      |         signlist = get_param([cb,'/Add'],'Inputs');
      |         set_param([cb,'/Add'],'Inputs',[signlist,'+']);
      |      catch 
      |      end
      | 
      | 
      |      try
      |          if rem(rowNo,6) ~= 0
      |         set_param([cb,'/Discrete FIR Filter ',num2str(i)],...
      |                   'Coefficients', [sprintf('transpose(squeeze(body.hydroForce.hf1.irkb(:,%d,%d)))',rem(rowNo,6),i)]); 
      |          elseif rem(rowNo,6) == 0
      |         set_param([cb,'/Discrete FIR Filter ',num2str(i)],...
      |                   'Coefficients', [sprintf('transpose(squeeze(body.hydroForce.hf1.irkb(:,%d,%d)))',6,i)]); 
      |          end
      |      catch
      |      end
      | 
      |      try
      |         add_line(cb,...
      |         ['Demux/',num2str(i)],...
      |         ['Discrete FIR Filter ',num2str(i),'/1'], ...     
      |         'autorouting','on');
      |      catch
      |      end
      | 
      | 
      |      try
      |         add_line(cb,...
      |         ['Discrete FIR Filter ',num2str(i),'/1'], ...     
      |         ['Add/', num2str(i)],...
      |         'autorouting','on');
      |     catch 
      |     end
      | end
  Gain : Gain  Gain=simu.cicDt
  Mux : Mux  Inputs=1
  Out1 : Outport
  wires:
  Gain/1 -> Out1/1
  FIR_filter_row/1(Out1) -> Mux/1
  velocity/1 -> FIR_filter_row/1(In1)
  Mux/1 -> Gain/1

== system WECSim_Lib_Body_Elements/Rigid Body/Hydrodynamic Body/Hydrostatic Restoring Force Calculation/Linear and Nonlinear Restoring Force Variant Subsystem/Linear Hydrostatic Restoring Force/Net Buoyancy Force ==
  note: The total buoyancy force is due to the vertical buoyancy force (gravity - buoyancy) and a rotational buoyancy force if the center of gravity is not aligned with the center of buoyancy.
      |
      | F_NetBuoyancy = F_gravity - F_buoyancy + F_rotational_buoyancy
      |
      | F_rotational_buoyancy = (cb-cg) x F_buoyancy
      | F_buoyancy = rho*g*V_0
      | F_gravity = m*g
  Body Mass : Inport
  Volume : Inport  Port=2
  Center of Buoyancy : Inport  Port=3
  Add1 : Sum  Inputs=+-
  Add2 : Sum
  Add3 : Sum  Inputs=+-
  Assignment (Add Net Bouyancy Force to Z-Direction) : Assignment  IndexOptions=Index vector (dialog)  Indices=3  OutputSizes=1
  Assignment (Add Net Bouyancy Force to Z-Direction)1 : Assignment  IndexOptions=Index vector (dialog)  Indices=3  OutputSizes=1
  Assignment (Add Net Bouyancy Force to Z-Direction)2 : Assignment  IndexOptions=Index vector (dialog)  Indices=4:6  OutputSizes=1
  Center of Gravity : Constant  Value=body.centerGravity
  Constant1 : Constant  Value=zeros(1,body.dof)
  Constant2 : Constant  Value=[0 0 0]
  Cross Product : vrlib/Utilities/Cross Product
  Gravity : Constant  Value=simu.gravity
  Product : Product
  Product1 : Product  Inputs=3
  Water Density : Constant  Value=simu.rho
  F_NetBuoyancy : Outport
  wires:
  Assignment (Add Net Bouyancy Force to Z-Direction)2/1 -> Add2/2  "Rotational buoyancy force"
  Product/1 -> Add1/1  "F_Gravity"
  Product1/1 -> Add1/2, Assignment (Add Net Bouyancy Force to Z-Direction)1/2  "F_Buoyancy"
  Gravity/1 -> Product1/2, Product/1  "g"
  Water Density/1 -> Product1/1  "rho"
  Assignment (Add Net Bouyancy Force to Z-Direction)/1 -> Add2/1  "Vertical Buoyancy Force"
  Assignment (Add Net Bouyancy Force to Z-Direction)1/1 -> Cross Product/1
  Constant1/1 -> Assignment (Add Net Bouyancy Force to Z-Direction)2/1, Assignment (Add Net Bouyancy Force to Z-Direction)/1
  Center of Gravity/1 -> Add3/2  "cg"
  Constant2/1 -> Assignment (Add Net Bouyancy Force to Z-Direction)1/1
  Add3/1 -> Cross Product/2
  Add2/1 -> F_NetBuoyancy/1  "Net buoyancy force"
  Cross Product/1 -> Assignment (Add Net Bouyancy Force to Z-Direction)2/2
  Body Mass/1 -> Product/2  "m"
  Add1/1 -> Assignment (Add Net Bouyancy Force to Z-Direction)/2
  Volume/1 -> Product1/3  "V0"
  Center of Buoyancy/1 -> Add3/1  "cb"

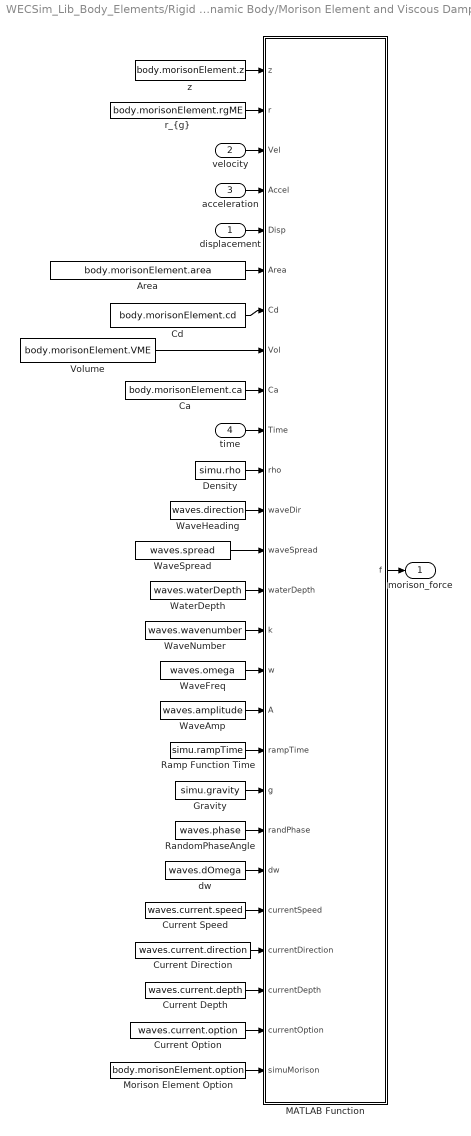
== system WECSim_Lib_Body_Elements/Rigid Body/Hydrodynamic Body/Morison Element and Viscous Damping Force Calculation/Morison Element Variant Subsystem/Morison Element On/Irregular Wave Morison Force ==
  displacement : Inport
  velocity : Inport  Port=2
  acceleration : Inport  Port=3
  time : Inport  Port=4
  Area : Constant  Value=body.morisonElement.area  VectorParams1D=off
  Ca : Constant  Value=body.morisonElement.ca  VectorParams1D=off
  Cd : Constant  Value=body.morisonElement.cd  VectorParams1D=off
  Current Depth : Constant  Value=waves.current.depth
  Current Direction : Constant  Value=waves.current.direction
  Current Option : Constant  Value=waves.current.option
  Current Speed : Constant  Value=waves.current.speed
  Density : Constant  Value=simu.rho
  Gravity : Constant  Value=simu.gravity
  MATLAB Function : MATLAB Function  TreatAsAtomicUnit=on
  Morison Element Option : Constant  Value=body.morisonElement.option
  Ramp Function Time : Constant  Value=simu.rampTime
  RandomPhaseAngle : Constant  Value=waves.phase  VectorParams1D=off
  Volume : Constant  Value=body.morisonElement.VME  VectorParams1D=off
  WaterDepth : Constant  Value=waves.waterDepth
  WaveAmp : Constant  Value=waves.amplitude
  WaveFreq : Constant  Value=waves.omega
  WaveHeading : Constant  Value=waves.direction
  WaveNumber : Constant  Value=waves.wavenumber
  WaveSpread : Constant  Value=waves.spread
  dw : Constant  Value=waves.dOmega  VectorParams1D=off
  "r_{g}" : Constant  Value=body.morisonElement.rgME  VectorParams1D=off
  z : Constant  Value=body.morisonElement.z  VectorParams1D=off
  morison_force : Outport
  wires:
  MATLAB Function/1(f) -> morison_force/1
  z/1 -> MATLAB Function/1(z)
  "r_{g}"/1 -> MATLAB Function/2(r)
  velocity/1 -> MATLAB Function/3(Vel)
  acceleration/1 -> MATLAB Function/4(Accel)
  displacement/1 -> MATLAB Function/5(Disp)
  Area/1 -> MATLAB Function/6(Area)
  Cd/1 -> MATLAB Function/7(Cd)
  Volume/1 -> MATLAB Function/8(Vol)
  Ca/1 -> MATLAB Function/9(Ca)
  time/1 -> MATLAB Function/10(Time)
  Density/1 -> MATLAB Function/11(rho)
  WaveHeading/1 -> MATLAB Function/12(waveDir)
  WaterDepth/1 -> MATLAB Function/14(waterDepth)
  WaveNumber/1 -> MATLAB Function/15(k)
  WaveFreq/1 -> MATLAB Function/16(w)
  WaveAmp/1 -> MATLAB Function/17(A)
  Ramp Function Time/1 -> MATLAB Function/18(rampTime)
  Gravity/1 -> MATLAB Function/19(g)
  RandomPhaseAngle/1 -> MATLAB Function/20(randPhase)
  dw/1 -> MATLAB Function/21(dw)
  Current Speed/1 -> MATLAB Function/22(currentSpeed)
  Current Direction/1 -> MATLAB Function/23(currentDirection)
  Current Depth/1 -> MATLAB Function/24(currentDepth)
  Current Option/1 -> MATLAB Function/25(currentOption)
  Morison Element Option/1 -> MATLAB Function/26(simuMorison)
  WaveSpread/1 -> MATLAB Function/13(waveSpread)

== system WECSim_Lib_Body_Elements/Rigid Body/Hydrodynamic Body/Morison Element and Viscous Damping Force Calculation/Morison Element Variant Subsystem/Morison Element On/No Wave Morison Force ==
  displacement : Inport
  velocity : Inport  Port=2
  acceleration : Inport  Port=3
  time : Inport  Port=4
  Area : Constant  Value=body.morisonElement.area  VectorParams1D=off
  Ca : Constant  Value=body.morisonElement.ca  VectorParams1D=off
  Cd : Constant  Value=body.morisonElement.cd  VectorParams1D=off
  Current Depth : Constant  Value=waves.current.depth
  Current Direction : Constant  Value=waves.current.direction
  Current Option : Constant  Value=waves.current.option
  Current Speed : Constant  Value=waves.current.speed
  Density : Constant  Value=simu.rho
  Morison Element Option : Constant  Value=body.morisonElement.option
  MorisonElement(s) : MATLAB Function  TreatAsAtomicUnit=on
  Ramp Function Time : Constant  Value=simu.rampTime
  Volume : Constant  Value=body.morisonElement.VME  VectorParams1D=off
  "r_{g}" : Constant  Value=body.morisonElement.rgME  VectorParams1D=off
  z : Constant  Value=body.morisonElement.z  VectorParams1D=off
  morison_force : Outport
  wires:
  MorisonElement(s)/1(f) -> morison_force/1
  z/1 -> MorisonElement(s)/1(z)
  "r_{g}"/1 -> MorisonElement(s)/2(r)
  velocity/1 -> MorisonElement(s)/3(Vel)
  acceleration/1 -> MorisonElement(s)/4(Accel)
  displacement/1 -> MorisonElement(s)/5(Disp)
  Area/1 -> MorisonElement(s)/6(Area)
  Cd/1 -> MorisonElement(s)/7(Cd)
  Volume/1 -> MorisonElement(s)/8(Vol)
  Ca/1 -> MorisonElement(s)/9(Ca)
  time/1 -> MorisonElement(s)/10(Time)
  Density/1 -> MorisonElement(s)/11(rho)
  Ramp Function Time/1 -> MorisonElement(s)/12(rampTime)
  Current Speed/1 -> MorisonElement(s)/13(currentSpeed)
  Current Direction/1 -> MorisonElement(s)/14(currentDirection)
  Current Depth/1 -> MorisonElement(s)/15(currentDepth)
  Current Option/1 -> MorisonElement(s)/16(currentOption)
  Morison Element Option/1 -> MorisonElement(s)/17(bodyMorison)
